simulink model "zakladny_model_jcbm"  (R2026b)
settings: Solver=FixedStepAuto  StopTime=10  FixedStep=0.00001
values from neighbouring files (symbols this model uses):
  cfi = (Ua-Ra*I)/w    (= 1.37353129893)    [vypocty_pre_studentov.m]
  I = 121    [vypocty_pre_studentov.m]
  J = 6*JM    (= 1.74)    [vypocty_pre_studentov.m]
  Ka = 1/Ra    (= 7.63358778626)    [vypocty_pre_studentov.m]
  KI = 10/Imax    (= 0.0413223140496)    [vypocty_pre_studentov.m]
  Kr = Ta/(2*Ttm*Ktm*Ka*KI)    (= 0.0484)    [vypocty_pre_studentov.m]
  KRw = J*KI/(2*(2*Ttm)*cfi*Kw)    (= 154.027501383)    [vypocty_pre_studentov.m]
  Ktm = 100    [vypocty_pre_studentov.m]
  Kw = 10/(2*w)    (= 0.0169928825623)    [vypocty_pre_studentov.m]
  Ta = La/Ra    (= 0.0152671755725)    [vypocty_pre_studentov.m]
  Ti = TR/Kr    (= 0.315437511829)    [vypocty_pre_studentov.m]
  TIw = TRw/KRw    (= 0.0002596938835)    [vypocty_pre_studentov.m]
  Ttm = 0.005    [vypocty_pre_studentov.m]
  w = n/9.55    (= 294.240837696)    [vypocty_pre_studentov.m]
libraries: SignalEditorBlockLib x1
settings Model: SimulationMode=accelerator  Creator=Peter  LastModifiedBy=patrikmitro
settings RTWCC: GPUComputeCapability=5.0

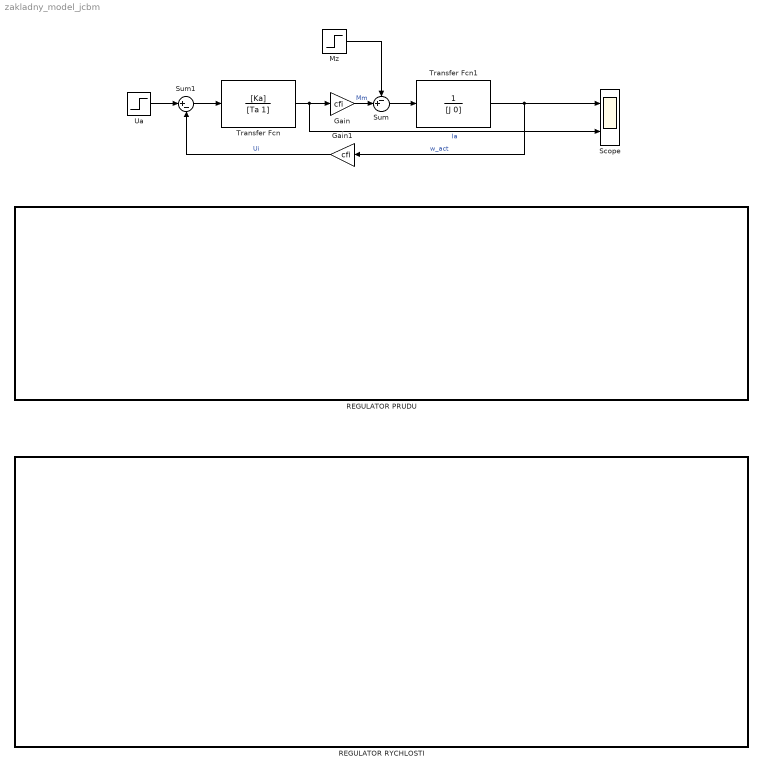
== system zakladny_model_jcbm ==
  Gain : Gain  Gain=cfi
  Gain1 : Gain  Gain=cfi
  Mz : Step  Time=1.5  FinalValue=M  SampleTime=0
  REGULATOR PRUDU : Subsystem
  REGULATOR RYCHLOSTI : Subsystem
  Scope : Scope  NumInputPorts=2
      settings: ActiveDisplayYMinimum=-38.222494745343575  ActiveDisplayYMaximum=344.00245270809222
  Sum : Sum  Inputs=-+|
  Sum1 : Sum  Inputs=|+-
  Transfer Fcn : TransferFcn  Numerator=[Ka]  Denominator=[Ta 1]
  Transfer Fcn1 : TransferFcn  Denominator=[J 0]
  Ua : Step  Time=0.2  FinalValue=Ua  SampleTime=0
  wires:
  Transfer Fcn/1 -> Scope/2, Gain/1  "Ia"
  Sum1/1 -> Transfer Fcn/1
  Gain/1 -> Sum/2  "Mm"
  Sum/1 -> Transfer Fcn1/1
  Transfer Fcn1/1 -> Gain1/1, Scope/1  "w_act"
  Gain1/1 -> Sum1/2  "Ui"
  Ua/1 -> Sum1/1
  Mz/1 -> Sum/1

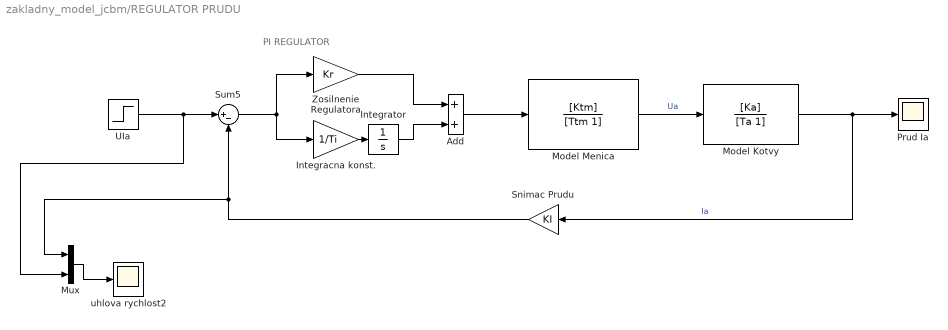
== system zakladny_model_jcbm/REGULATOR PRUDU ==
  note: PI REGULATOR
  Add : Sum
  Integracna konst. : Gain  Gain=1/Ti
  Integrator : Integrator
  Model Kotvy : TransferFcn  Numerator=[Ka]  Denominator=[Ta 1]
  Model Menica : TransferFcn  Numerator=[Ktm]  Denominator=[Ttm 1]
  Mux : Mux  Inputs=2
  Prud Ia : Scope
      settings: ActiveDisplayYMinimum=-15.778610405656929  ActiveDisplayYMaximum=142.00749365091238  DataLoggingVariableName=ScopeData2
  Snimac Prudu : Gain  Gain=KI
  Sum5 : Sum  Inputs=|+-
  UIa : Step  Time=0  FinalValue=KI*I  SampleTime=0
  Zosilnenie Regulatora : Gain  Gain=Kr
  uhlova rychlost2 : Scope
      settings: ActiveDisplayYMinimum=4.7802760280457228  ActiveDisplayYMaximum=5.2371776000642791  YLabel=Napätie [V]  DataLoggingVariableName=ScopeData9
  wires:
  Integrator/1 -> Add/2
  Model Menica/1 -> Model Kotvy/1  "Ua"
  Zosilnenie Regulatora/1 -> Add/1
  Integracna konst./1 -> Integrator/1
  Add/1 -> Model Menica/1
  Model Kotvy/1 -> Prud Ia/1, Snimac Prudu/1  "Ia"
  Sum5/1 -> Zosilnenie Regulatora/1, Integracna konst./1
  Mux/1 -> uhlova rychlost2/1
  UIa/1 -> Mux/2, Sum5/1
  Snimac Prudu/1 -> Mux/1, Sum5/2

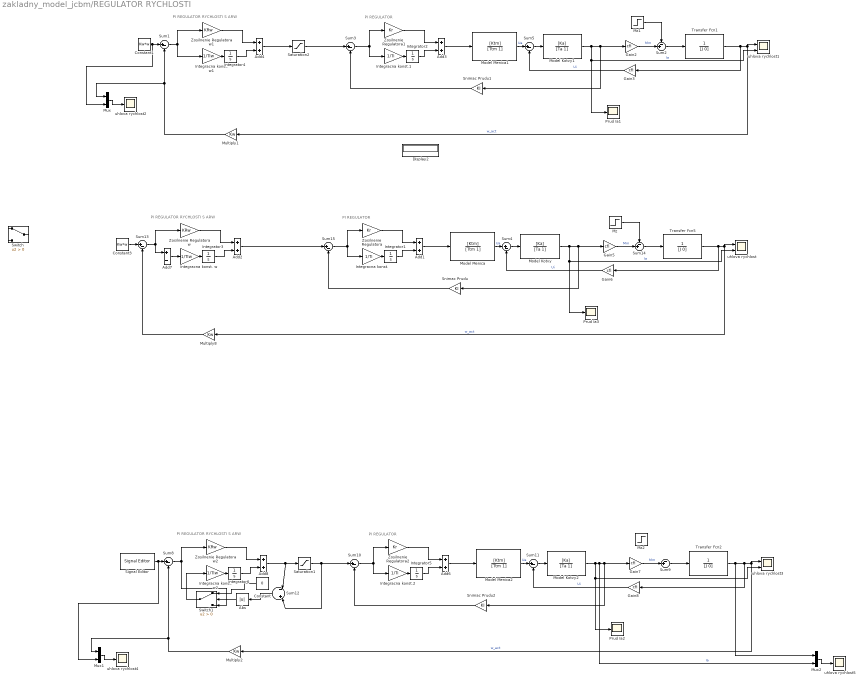
== system zakladny_model_jcbm/REGULATOR RYCHLOSTI ==
  note: PI REGULATOR RYCHLOSTI S ARW
  note: PI REGULATOR
  note: PI REGULATOR RYCHLOSTI S ARW
  note: PI REGULATOR
  note: PI REGULATOR RYCHLOSTI S ARW
  note: PI REGULATOR
  Abs : Abs  SaturateOnIntegerOverflow=off
  Add{1..4,6,8} (6 alike) : Sum
  Add7 : Sum  Inputs=+-
  Constant : Constant  Value=0
  Constant1 : Constant  Value=Kw*w
  Constant3 : Constant  Value=Kw*w
  Display2 : Display
  Gain{2..3,5..8} (6 alike) : Gain  Gain=cfi
  Integracna konst. : Gain  Gain=1/Ti
  Integracna konst. w : Gain  Gain=1/TIw
  Integracna konst. w1 : Gain  Gain=1/TIw
  Integracna konst. w2 : Gain  Gain=1/TIw
  Integracna konst.1 : Gain  Gain=1/Ti
  Integracna konst.2 : Gain  Gain=1/Ti
  Integrator{1..6} (6 alike) : Integrator
  Model Kotvy : TransferFcn  Numerator=[Ka]  Denominator=[Ta 1]
  Model Kotvy1 : TransferFcn  Numerator=[Ka]  Denominator=[Ta 1]
  Model Kotvy2 : TransferFcn  Numerator=[Ka]  Denominator=[Ta 1]
  Model Menica : TransferFcn  Numerator=[Ktm]  Denominator=[Ttm 1]
  Model Menica1 : TransferFcn  Numerator=[Ktm]  Denominator=[Ttm 1]
  Model Menica2 : TransferFcn  Numerator=[Ktm]  Denominator=[Ttm 1]
  Multiply1 : Gain  Gain=Kw
  Multiply2 : Gain  Gain=Kw
  Multiply8 : Gain  Gain=Kw
  Mux : Mux  Inputs=2
  Mux1 : Mux  Inputs=2
  Mux2 : Mux  Inputs=2
  Mz : Step  Time=6  FinalValue=M  SampleTime=0
  Mz1 : Step  Time=3  FinalValue=M  SampleTime=0
  Mz2 : Step  Time=0  FinalValue=M  SampleTime=0
  Prud Ia1 : Scope
      settings: ActiveDisplayYMinimum=-6.304744121650419  ActiveDisplayYMaximum=40.7951978129335
  Prud Ia2 : Scope
      settings: ActiveDisplayYMinimum=-324.06712341968972  ActiveDisplayYMaximum=323.86806741485458  DataLoggingVariableName=ScopeData5
  Prud Ia3 : Scope
      settings: ActiveDisplayYMinimum=-324.06712341968972  ActiveDisplayYMaximum=323.86806741485458  DataLoggingVariableName=ScopeData7
  Saturation1 : Saturate  UpperLimit=10  LowerLimit=-10
  Saturation2 : Saturate  UpperLimit=10  LowerLimit=-10
  Signal Editor : SignalEditorBlockLib/Signal Editor  FileName=untitled.mat  ActiveScenario=Scenario  ActiveSignal=Signal 1  IsBus=off  OutputBusObjectStr=Bus: BusObject  SampleTime=0  ZeroCross=off  OutputAfterFinalValue=Setting to zero  Unit=inherit  PreserveSignalName=on  ApplySigPropsToAllScenarios=off  ApplySigPropsToAllSignals=off  SignalPropertySource=Signal data in MAT file
  Snimac Prudu : Gain  Gain=KI
  Snimac Prudu1 : Gain  Gain=KI
  Snimac Prudu2 : Gain  Gain=KI
  Sum{1,3..5,8,10..11,13,15} (9 alike) : Sum  Inputs=|+-
  Sum12 : Sum  Inputs=|-||+|
  Sum14 : Sum  Inputs=-+|
  Sum2 : Sum  Inputs=-+|
  Sum9 : Sum  Inputs=-+|
  Switch : Switch  Criteria=u2 > Threshold  SaturateOnIntegerOverflow=off  InputSameDT=off
  Switch1 : Switch  Criteria=u2 > Threshold  SaturateOnIntegerOverflow=off  InputSameDT=off
  Transfer Fcn1 : TransferFcn  Denominator=[J 0]
  Transfer Fcn2 : TransferFcn  Denominator=[J 0]
  Transfer Fcn5 : TransferFcn  Denominator=[J 0]
  Zosilnenie Regulatora : Gain  Gain=Kr
  Zosilnenie Regulatora w : Gain  Gain=KRw
  Zosilnenie Regulatora w1 : Gain  Gain=KRw
  Zosilnenie Regulatora w2 : Gain  Gain=KRw
  Zosilnenie Regulatora1 : Gain  Gain=Kr
  Zosilnenie Regulatora2 : Gain  Gain=Kr
  uhlova rychlost : Scope  NumInputPorts=2
      settings: ActiveDisplayYMinimum=-52.980670595871537  ActiveDisplayYMaximum=476.826035362844  DataLoggingVariableName=ScopeData6
  uhlova rychlost1 : Scope  NumInputPorts=2
      settings: ActiveDisplayYMinimum=-54.618373699353263  ActiveDisplayYMaximum=491.56536329417952  DataLoggingVariableName=ScopeData3
  uhlova rychlost2 : Scope
      settings: ActiveDisplayYMinimum=-1.0239948076243768  ActiveDisplayYMaximum=11.113760726959164  YLabel=Napätie [V]  DataLoggingVariableName=ScopeData4
  uhlova rychlost3 : Scope  NumInputPorts=2
      settings: ActiveDisplayYMinimum=-36.904963795985744  ActiveDisplayYMaximum=332.14467416387174  DataLoggingVariableName=ScopeData8
  uhlova rychlost4 : Scope
      settings: ActiveDisplayYMinimum=-6.2852217576583183  ActiveDisplayYMaximum=6.2769211567125263  YLabel=Napätie [V]  DataLoggingVariableName=ScopeData10
  uhlova rychlost5 : Scope
      settings: ActiveDisplayYMinimum=-369.20501943672582  ActiveDisplayYMaximum=369.311000796611  YLabel=Napätie [V]  DataLoggingVariableName=ScopeData11
  wires:
  Integrator1/1 -> Add1/2
  Zosilnenie Regulatora/1 -> Add1/1
  Integracna konst. w/1 -> Integrator3/1
  Sum14/1 -> Transfer Fcn5/1
  Add2/1 -> Sum15/1
  Transfer Fcn5/1 -> Gain6/1, Multiply8/1, uhlova rychlost/1  "w_act"
  Gain6/1 -> Sum4/2  "Ui"
  Integracna konst./1 -> Integrator1/1
  Gain5/1 -> Sum14/2  "Mm"
  Model Kotvy/1 -> uhlova rychlost/2, Prud Ia3/1, Gain5/1, Snimac Prudu/1  "Ia"
  Sum15/1 -> Zosilnenie Regulatora/1, Integracna konst./1
  Model Menica/1 -> Sum4/1  "Ua"
  Add1/1 -> Model Menica/1
  Sum4/1 -> Model Kotvy/1
  Sum13/1 -> Zosilnenie Regulatora w/1, Add7/1
  Snimac Prudu/1 -> Sum15/2
  Integrator3/1 -> Add2/2
  Add7/1 -> Integracna konst. w/1
  Zosilnenie Regulatora w/1 -> Add2/1
  Constant3/1 -> Sum13/1
  Add3/1 -> Model Menica1/1
  Sum1/1 -> Integracna konst. w1/1, Zosilnenie Regulatora w1/1
  Integracna konst. w1/1 -> Integrator4/1
  Zosilnenie Regulatora1/1 -> Add3/1
  Constant1/1 -> Mux/2, Sum1/1
  Snimac Prudu1/1 -> Sum3/2
  Integrator2/1 -> Add3/2
  Gain2/1 -> Sum2/2  "Mm"
  Gain3/1 -> Sum5/2  "Ui"
  Zosilnenie Regulatora w1/1 -> Add4/1
  Sum3/1 -> Zosilnenie Regulatora1/1, Integracna konst.1/1
  Model Kotvy1/1 -> uhlova rychlost1/2, Prud Ia1/1, Gain2/1, Snimac Prudu1/1  "Ia"
  Integracna konst.1/1 -> Integrator2/1
  Sum5/1 -> Model Kotvy1/1
  Sum2/1 -> Transfer Fcn1/1
  Multiply1/1 -> Mux/1, Sum1/2
  Transfer Fcn1/1 -> Gain3/1, Multiply1/1, uhlova rychlost1/1  "w_act"
  Model Menica1/1 -> Sum5/1  "Ua"
  Integrator4/1 -> Add4/2
  Mux/1 -> uhlova rychlost2/1
  Add6/1 -> Model Menica2/1
  Sum12/1 -> Abs/1
  Sum8/1 -> Switch1/3, Zosilnenie Regulatora w2/1
  Integracna konst. w2/1 -> Integrator6/1
  Add8/1 -> Saturation1/1, Sum12/1
  Zosilnenie Regulatora2/1 -> Add6/1
  Snimac Prudu2/1 -> Sum10/2
  Integrator5/1 -> Add6/2
  Gain7/1 -> Sum9/2  "Mm"
  Saturation1/1 -> Sum12/2, Sum10/1
  Gain8/1 -> Sum11/2  "Ui"
  Zosilnenie Regulatora w2/1 -> Add8/1
  Sum10/1 -> Zosilnenie Regulatora2/1, Integracna konst.2/1
  Model Kotvy2/1 -> uhlova rychlost3/2, Prud Ia2/1, Mux2/2, Gain7/1, Snimac Prudu2/1  "Ia"
  Integracna konst.2/1 -> Integrator5/1
  Sum11/1 -> Model Kotvy2/1
  Sum9/1 -> Transfer Fcn2/1
  Transfer Fcn2/1 -> Mux2/1, Gain8/1, Multiply2/1, uhlova rychlost3/1  "w_act"
  Model Menica2/1 -> Sum11/1  "Ua"
  Integrator6/1 -> Add8/2
  Abs/1 -> Switch1/2
  Switch1/1 -> Integracna konst. w2/1
  Constant/1 -> Switch1/1
  Multiply8/1 -> Sum13/2
  Add4/1 -> Saturation2/1
  Mz/1 -> Sum14/1
  Saturation2/1 -> Sum3/1
  Mz1/1 -> Sum2/1
  Mux1/1 -> uhlova rychlost4/1
  Signal Editor/1 -> Mux1/2, Sum8/1
  Multiply2/1 -> Sum8/2, Mux1/1
  Mux2/1 -> uhlova rychlost5/1
